simulink model "M2_LoadInjection_P05"  (R2025b)
settings: Solver=VariableStepAuto  StartTime=0.0  StopTime=30  RelTol=1e-3  AbsTol=1e-3  EnableMultiTasking=on
model workspace (MAT data in the model file):
  A_d4 = 2
  A_q3 = 15
  B_d4 = 8.75
  B_q3 = 45
  F0_x = 0
  F0_y = 100000
  omega_F = 0.698131700798
  omega_traj = 0.314159265359
undefined symbols (not defined in the file): X, Y, Z
libraries: nesl_utility x12, sm_lib x9
Description:
  | MS02P05 copy built by build_M2_LoadInjection_P05.m from M2_LoadInjection.slx (MD5 f17dcb99da107e28bae416fc79d4f5ec) on 2026-11-18 14:56. Only change: handle-angle Sine Wave Amplitude/Bias read A_q3/B_q3 [deg] (model-workspace defaults 15/45). Do not edit by hand; rebuild with the builder.
settings Model: Creator=Mritunjoy Hazra  LastModifiedBy=IIT KGP
settings SolverCC: AutoScaleAbsTol=off  AlgebraicLoopSolver=TrustRegion  MaxZcPerStep=1.0
settings DataIOCC: LimitDataPoints=on  MaxDataPoints=10000  OutputOption=SpecifiedOutputTimes  OutputTimes=0:0.01:30
settings OptimizationCC: ReuseModelBlockBuffer=off  LifeSpan=inf
settings DebuggingCC: UnconnectedInputMsg=warning  UnconnectedOutputMsg=warning  UnconnectedLineMsg=warning  AllowSymbolicDim=off  SubsystemReferenceDiagnosticForUnitTest=warning  SFUnexpectedBacktrackingDiag=warning  SFNoUnconditionalDefaultTransitionDiag=warning  SFExecutionAtInitializationDiag=none  ArithmeticOperatorsInVariantConditions=warning
settings ModelReferenceCC: EnableRefExpFcnMdlSchedulingChecks=on
settings SFSimCC: SimUseLocalCustomCode=off  CustomCodeUndefinedFunction=UseInterfaceOnly
settings RTWCC: RTWUseLocalCustomCode=off  GPUComputeCapability=3.5  DLArmComputeVersion=19.05
settings CodeAppCC: StateflowObjectComments=on
settings GRTTargetCC: TargetLangStandard=C89/C90 (ANSI)
settings ConfigComp: CovMetricSettings=dw  CovSaveCumulativeToWorkspaceVar=on  CovSaveSingleToWorkspaceVar=on  CovExternalEMLEnable=off  CovSFcnEnable=off
settings SimscapeCC: SimscapeLogType=all  SimscapeLogSimulationStatistics=on  SimscapeLogDataHistory=10000.0

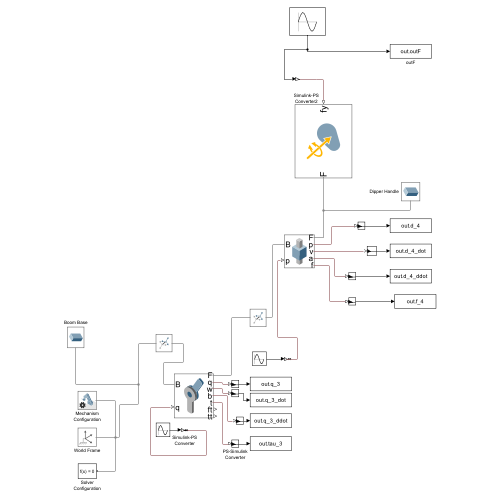
[thumbnail: Simulink's stored preview of the top-level diagram]
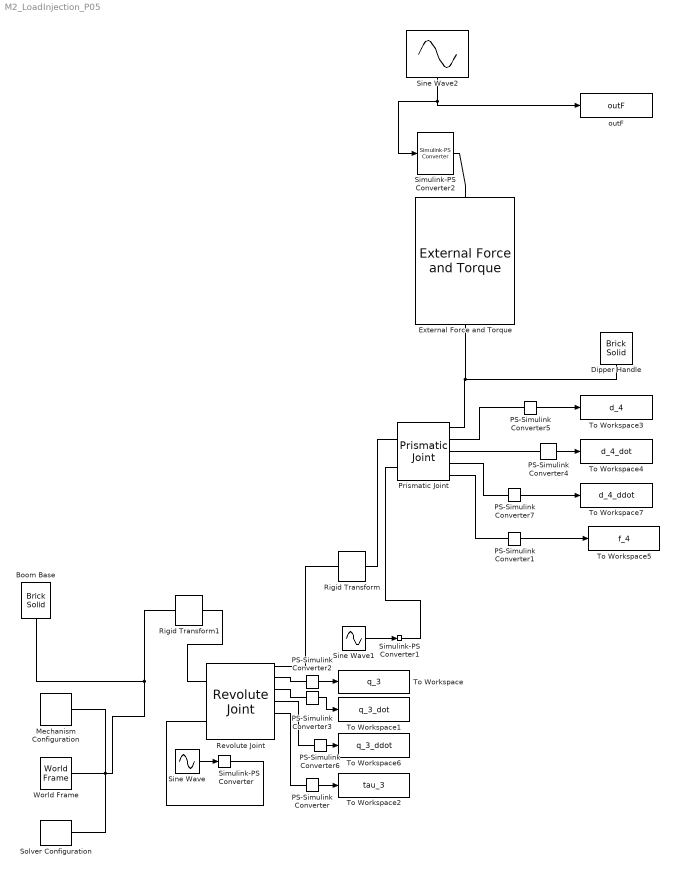
== system M2_LoadInjection_P05 ==
  Boom Base : sm_lib/Body Elements/Brick Solid  BrickDimensions=[1 1 1]  BrickDimensionsUnits=m  ExportEntireGeometry=off  InertiaType=Custom  BasedOnType=Density  Density=1000  DensityUnits=kg/m^3  Mass=135000  MassUnits=kg  CenterOfMass=[8 0 0]  CenterOfMassUnits=m  MomentsOfInertia=[0 0 2500000]  MomentsOfInertiaUnits=kg*m^2  ProductsOfInertia=[0 0 0]  ProductsOfInertiaUnits=kg*m^2  GraphicType=FromGeometry  MarkerShape=Sphere  MarkerSize=10  GraphicVisPropType=SimpleVisualProperties  GraphicDiffuseColor=[0.5 0.5 0.5]  GraphicOpacity=1.0  GraphicSpecularColor=[0.5 0.5 0.5 1.0]  GraphicAmbientColor=[0.15 0.15 0.15 1.0]  GraphicEmissiveColor=[0.0 0.0 0.0 1.0]  GraphicShininess=75  DoExposeReferenceFrame=on  SerializedFrames=<Frames/>
  Dipper Handle : sm_lib/Body Elements/Brick Solid  BrickDimensions=[1 1 1]  BrickDimensionsUnits=m  ExportEntireGeometry=off  InertiaType=Custom  BasedOnType=Density  Density=1000  DensityUnits=kg/m^3  Mass=[54300]  MassUnits=kg  CenterOfMass=[0 0 -2.82]  CenterOfMassUnits=m  MomentsOfInertia=[287900 0 0 ]  MomentsOfInertiaUnits=kg*m^2  ProductsOfInertia=[0 0 0]  ProductsOfInertiaUnits=kg*m^2  GraphicType=FromGeometry  MarkerShape=Sphere  MarkerSize=10  GraphicVisPropType=SimpleVisualProperties  GraphicDiffuseColor=[0.5 0.5 0.5]  GraphicOpacity=1  GraphicSpecularColor=[0.5 0.5 0.5 1.0]  GraphicAmbientColor=[0.15 0.15 0.15 1.0]  GraphicEmissiveColor=[0.0 0.0 0.0 1.0]  GraphicShininess=75  DoExposeReferenceFrame=on  SerializedFrames=<Frames/>
  External Force and Torque : sm_lib/Forces and Torques/External Force and Torque  EnableForceX=off  EnableForceY=on  EnableForceZ=off  EnableForce=off  ForceResolutionFrame=World  EnableTorqueX=off  EnableTorqueY=off  EnableTorqueZ=off  EnableTorque=off  TorqueResolutionFrame=AttachedFrame
  Mechanism Configuration : sm_lib/Utilities/Mechanism Configuration  UniformGravity=Constant  GravityVector=[0 -9.80665 0]  GravityVectorUnits=m/s^2  LinearizationDelta=0.001  JointModeTransitionNonlinearIterations=2
  PS-Simulink Converter{,1..7} (8 alike) : nesl_utility/PS-Simulink Converter  PhysicalDomain=network_engine_domain  SubClassName=ps_output  LeftPortType=input  RightPortType=output  PseudoPeriodic=off  Frequencies=[]  VectorFormat=inherit  Unit=inherit  AffineConversion=off
  Prismatic Joint : sm_lib/Joints/Prismatic Joint  JointMode=Normal  CompositeWrenchDir=FollowerOnBase  CompositeWrenchFrame=BaseFrame  SenseConstraintForce=off  SenseConstraintTorque=off  SenseTotalForce=off  SenseTotalTorque=off  PositionTargetSpecify=off  PositionTargetPriority=High  PositionTargetValue=0  PositionTargetValueUnits=m  VelocityTargetSpecify=off  VelocityTargetPriority=High  VelocityTargetValue=0  VelocityTargetValueUnits=m/s  EquilibriumPosition=0  EquilibriumPositionUnits=m  SpringStiffness=0  SpringStiffnessUnits=N/m  DampingCoefficient=1473.0  DampingCoefficientUnits=N/(m/s)  LowerLimitSpecify=off  LowerLimitBound=-1  LowerLimitBoundUnits=m  LowerLimitStiffness=1e6  LowerLimitStiffnessUnits=N/m  LowerLimitDamping=1e3  LowerLimitDampingUnits=N/(m/s)  LowerLimitTransitionRegionWidth=1e-4  LowerLimitTransitionRegionWidthUnits=m  UpperLimitSpecify=off  UpperLimitBound=1  UpperLimitBoundUnits=m  UpperLimitStiffness=1e6  UpperLimitStiffnessUnits=N/m  UpperLimitDamping=1e3  UpperLimitDampingUnits=N/(m/s)  UpperLimitTransitionRegionWidth=1e-4  UpperLimitTransitionRegionWidthUnits=m  TorqueActuationMode=ComputedTorque  MotionActuationMode=InputMotion  SensePosition=on  SenseVelocity=on  SenseAcceleration=on  SenseTorqueForce=on  SenseLowerLimitTorqueForce=off  SenseUpperLimitTorqueForce=off
  Revolute Joint : sm_lib/Joints/Revolute Joint  JointMode=Normal  CompositeWrenchDir=FollowerOnBase  CompositeWrenchFrame=BaseFrame  SenseConstraintForce=off  SenseConstraintTorque=off  SenseTotalForce=on  SenseTotalTorque=on  PositionTargetSpecify=on  PositionTargetPriority=High  PositionTargetValue=30  PositionTargetValueUnits=deg  VelocityTargetSpecify=off  VelocityTargetPriority=High  VelocityTargetValue=0  VelocityTargetValueUnits=deg/s  EquilibriumPosition=0  EquilibriumPositionUnits=deg  SpringStiffness=0  SpringStiffnessUnits=N*m/deg  DampingCoefficient=66.322512  DampingCoefficientUnits=N*m/(deg/s)  LowerLimitSpecify=off  LowerLimitBound=-90  LowerLimitBoundUnits=deg  LowerLimitStiffness=1e4  LowerLimitStiffnessUnits=N*m/deg  LowerLimitDamping=10  LowerLimitDampingUnits=N*m/(deg/s)  LowerLimitTransitionRegionWidth=0.1  LowerLimitTransitionRegionWidthUnits=deg  UpperLimitSpecify=off  UpperLimitBound=90  UpperLimitBoundUnits=deg  UpperLimitStiffness=1e4  UpperLimitStiffnessUnits=N*m/deg  UpperLimitDamping=10  UpperLimitDampingUnits=N*m/(deg/s)  UpperLimitTransitionRegionWidth=0.1  UpperLimitTransitionRegionWidthUnits=deg  TorqueActuationMode=ComputedTorque  MotionActuationMode=InputMotion  SensePosition=on  SenseVelocity=on  SenseAcceleration=on  SenseTorqueForce=on  SenseLowerLimitTorqueForce=off  SenseUpperLimitTorqueForce=off
  Rigid Transform : sm_lib/Frames and Transforms/Rigid Transform  RotationMethod=StandardAxis  FollAlignAxisA=+X  BaseAlignAxisA=+Y  FollAlignAxisB=+Y  BaseAlignAxisB=+Z  RotationStandardAxis=+Y  RotationAngle=90  RotationAngleUnits=deg  RotationArbitraryAxis=[0 0 1]  RotationSequenceAxes=FollowerAxes  RotationSequence=XYX  RotationSequenceAngles=[0 0 0]  RotationSequenceAnglesUnits=deg  RotationMatrix=[1 0 0;0 1 0;0 0 1]  Quaternion=[1 0 0 0]  TranslationMethod=Cartesian  TranslationCartesianOffset=[1.5 0 0]  TranslationCartesianOffsetUnits=m  TranslationStandardAxis=+Z  TranslationStandardOffset=0  TranslationStandardOffsetUnits=m  TranslationROffset=0  TranslationROffsetUnits=m  TranslationThetaOffset=0  TranslationThetaOffsetUnits=deg  TranslationZOffset=0  TranslationZOffsetUnits=m
  Rigid Transform1 : sm_lib/Frames and Transforms/Rigid Transform  RotationMethod=None  FollAlignAxisA=+X  BaseAlignAxisA=+Y  FollAlignAxisB=+Y  BaseAlignAxisB=+Z  RotationStandardAxis=+X  RotationAngle=90  RotationAngleUnits=deg  RotationArbitraryAxis=[0 0 1]  RotationSequenceAxes=FollowerAxes  RotationSequence=XYX  RotationSequenceAngles=[0 0 0]  RotationSequenceAnglesUnits=deg  RotationMatrix=[1 0 0;0 1 0;0 0 1]  Quaternion=[1 0 0 0]  TranslationMethod=Cartesian  TranslationCartesianOffset=[0 0 0]  TranslationCartesianOffsetUnits=m  TranslationStandardAxis=+Z  TranslationStandardOffset=0  TranslationStandardOffsetUnits=m  TranslationROffset=0  TranslationROffsetUnits=m  TranslationThetaOffset=0  TranslationThetaOffsetUnits=deg  TranslationZOffset=0  TranslationZOffsetUnits=m
  Simulink-PS Converter : nesl_utility/Simulink-PS Converter  PhysicalDomain=network_engine_domain  SubClassName=ps_input  LeftPortType=input  RightPortType=output  PseudoPeriodic=off  Frequencies=[]  NoiseDistribution=none  NoiseParameters=[]  Unit=deg  AffineConversion=off  FilteringAndDerivatives=filter  SimscapeFilterOrder=2  InputFilterTimeConstant=0.05  UdotUserProvided=0
  Simulink-PS Converter1 : nesl_utility/Simulink-PS Converter  PhysicalDomain=network_engine_domain  SubClassName=ps_input  LeftPortType=input  RightPortType=output  PseudoPeriodic=off  Frequencies=[]  NoiseDistribution=none  NoiseParameters=[]  Unit=m  AffineConversion=off  FilteringAndDerivatives=filter  SimscapeFilterOrder=2  InputFilterTimeConstant=0.05  UdotUserProvided=0
  Simulink-PS Converter2 : nesl_utility/Simulink-PS Converter  PhysicalDomain=network_engine_domain  SubClassName=ps_input  LeftPortType=input  RightPortType=output  PseudoPeriodic=off  Frequencies=[]  NoiseDistribution=none  NoiseParameters=[]  Unit=N  AffineConversion=off  FilteringAndDerivatives=zero  SimscapeFilterOrder=2  InputFilterTimeConstant=0.05  UdotUserProvided=0
  Sine Wave : Sin  Amplitude=A_q3  Bias=B_q3  Frequency=omega_traj  SampleTime=0
  Sine Wave1 : Sin  Amplitude=A_d4  Bias=B_d4  Frequency=omega_traj  SampleTime=0
  Sine Wave2 : Sin  Amplitude=F0_y  Frequency=omega_F  SampleTime=0
  Solver Configuration : nesl_utility/Solver Configuration  PhysicalDomain=network_engine_domain  SubClassName=solver  LeftPortType=input  RightPortType=generic  Tones=[]  Harmonics=[]  SimulateNoise=off  Profile=off  UseLocalSampling=off  EnableSwitchedLinearOptims=on  FrequencyDomain=off  UseCCode=off  RelTol=0.001  AbsTol=1e-06  MinStep=1e-09  ToWorkspace=off  RevertToSquareIcSolve=off  NumHomotopyIterations=100  PhasorMode=off  PhasorModeNumHarmonics=1  ConsistencySolver=NEWTON_XTOL_AFTER_FTOL  IndexReductionMethod=DerivativeReplacement  DoDC=off  ResidualTolerance=1e-09  ConsistencyTolSource=GLOBAL  ConsistencyAbsTol=0.001  ConsistencyRelTol=0.001  ConsistencyTolFactor=0.001  UseLocalSolver=off  LocalSolverChoice=NE_BACKWARD_EULER_ADVANCER  ResolveIndetEquations=on  FunctionEvalNumThread=1  LocalSolverSampleTime=0.001  DoFixedCost=off  MaxNonlinIter=3  MaxModeIter=2  ComputeImpulses=off  ImpulseIterations=2  LinearAlgebra=Sparse  LinearAlgebraNumThread=0  EquationFormulation=NE_TIME_EF  DelaysMemoryBudget=1024  AutomaticFiltering=on  FilteringTimeConstant=0.001  PartitionStorageMethod=AS_NEEDED  PartitionMemoryBudget=1024  PartitionMethod=FAST  MultibodyUseLocalSolver=off  MultibodyLocalSolverChoice=ODE1  MultibodyLocalSolverSampleTime=0.001
  To Workspace : ToWorkspace  VariableName=q_3  SampleTime=0.01
  To Workspace1 : ToWorkspace  VariableName=q_3_dot  SampleTime=0.01
  To Workspace2 : ToWorkspace  VariableName=tau_3  SampleTime=0.01
  To Workspace3 : ToWorkspace  VariableName=d_4  SampleTime=0.01
  To Workspace4 : ToWorkspace  VariableName=d_4_dot  SampleTime=0.01
  To Workspace5 : ToWorkspace  VariableName=f_4  SampleTime=0.01
  To Workspace6 : ToWorkspace  VariableName=q_3_ddot  SampleTime=0.01
  To Workspace7 : ToWorkspace  VariableName=d_4_ddot  SampleTime=0.01
  World Frame : sm_lib/Frames and Transforms/World Frame
  outF : ToWorkspace  VariableName=outF  SampleTime=0.01
  wires:
  Sine Wave/1 -> Simulink-PS Converter/1
  Sine Wave1/1 -> Simulink-PS Converter1/1
  PS-Simulink Converter1/1 -> To Workspace5/1
  PS-Simulink Converter2/1 -> To Workspace/1
  PS-Simulink Converter3/1 -> To Workspace1/1
  PS-Simulink Converter/1 -> To Workspace2/1
  PS-Simulink Converter4/1 -> To Workspace4/1
  PS-Simulink Converter5/1 -> To Workspace3/1
  PS-Simulink Converter6/1 -> To Workspace6/1
  PS-Simulink Converter7/1 -> To Workspace7/1
  Sine Wave2/1 -> Simulink-PS Converter2/1, outF/1
  connections:
  Boom Base/RConn1 -- Rigid Transform1/LConn1 -- Solver Configuration/RConn1 -- World Frame/RConn1 -- Mechanism Configuration/RConn1
  Simulink-PS Converter/RConn1 -- Revolute Joint/LConn2
  Revolute Joint/RConn5 -- PS-Simulink Converter/LConn1
  Revolute Joint/RConn1 -- Rigid Transform/LConn1
  Rigid Transform/RConn1 -- Prismatic Joint/LConn1
  Prismatic Joint/RConn1 -- External Force and Torque/RConn1 -- Dipper Handle/RConn1
  Revolute Joint/RConn2 -- PS-Simulink Converter2/LConn1
  Revolute Joint/RConn3 -- PS-Simulink Converter3/LConn1
  Prismatic Joint/RConn5 -- PS-Simulink Converter1/LConn1
  Prismatic Joint/RConn3 -- PS-Simulink Converter4/LConn1
  PS-Simulink Converter5/LConn1 -- Prismatic Joint/RConn2
  Rigid Transform1/RConn1 -- Revolute Joint/LConn1
  Revolute Joint/RConn4 -- PS-Simulink Converter6/LConn1
  Prismatic Joint/RConn4 -- PS-Simulink Converter7/LConn1
  Simulink-PS Converter1/RConn1 -- Prismatic Joint/LConn2
  External Force and Torque/LConn1 -- Simulink-PS Converter2/RConn1
